simulink library "lib_imuCal"  (Simulink 9.0)
settings: Solver=VariableStepAuto  StartTime=0.0  StopTime=10.0  RelTol=1e-3
undefined symbols (not defined in the file): g, toa_imuBasicOrient
libraries: lib_CATutils_Utilities_ApplyName_v2 x14, lib_imuCal x2, simulink_extras x2, lib_CATutils_Override x2
(part 2 of 2)

== matlab function imuCal Subsystem/imuCal ==
  data: resetLowerFlag input double; pitchOffset output double; resetRaiseFlag input double; calDirectionFlag input double; getPitchOffsetFlag input double; liftHeight input double; tiltHePress input double; tiltRePress input double; liftPress input double; imuX input double; imuY input double; imuZ input double; liftAngle input double; tiltExt input double; steerAngle input double; toa_appNumber input double; toa_tiltBoreDia input double; toa_tiltRodDia input double; toa_liftBoreDia input double; toa_tiltNumCyl input double; toa_toolBcLength input double; lumpedWeight output double
function [pitchOffset, lumpedWeight] = imuCal(...
    resetLowerFlag, resetRaiseFlag, calDirectionFlag, getPitchOffsetFlag, ...
    liftHeight, tiltHePress, tiltRePress, liftPress, ...
    imuX, imuY, imuZ, ...
    liftAngle, tiltExt, steerAngle, ...
    toa_appNumber, toa_tiltBoreDia, toa_tiltRodDia, toa_liftBoreDia, toa_tiltNumCyl, toa_toolBcLength)
% IMUCAL Calibrate IMU
%
% Collects data during CPM calibration and calculates an IMU pitch offset
% calibration value.
%
% Data is collected between the *_TRIGGER_HEIGHT lift heights during the
% slow loaded raise and slow loaded lower portion of the CPM cal.  Then, a
% brute force search for the correct IMU pitch cal value begins.  For
% candidate pitch values (which are an input into the TOA weighing math,
% the following occurs.
%
% Tip-Off Assist weighing math is applied to obtain a corresponding weight
% signal for both raise a lower.  The signals include friction.  A
% phaseless notch filter is applied to the weight signals to remove machine
% resonance. The raise and lower weight signals are then sampled at the
% lift angles specified by *_LA_SLOPE_POINTS.  The weights at the sample
% points are averaged to produce a frictionless weight at each lift angle.
% Finally, the slope of the lift angle vs. frictionless weight curve is
% calculated.
%
% The correct IMU pitch cal value will be the one whose corresponding slope
% is closest to zero, because the correct cal value should produce the same
% weight across the lift range.

% To enable some code paths that may be useful for development.
DEBUG = false;

% Sample time
% Important for phaseless filtering
Ts = single(0.020);

% Constants
% Slope points a grid of lift angles (in degrees) that we sample the
% time-series data to for purposes of calculating slope efficiently.  This
% is done after phaseless filtering.
LA_SLOPE_POINTS_BOTTOM = -10;   % MUST be higher than BOTTOM_TRIGGER_HEIGHT
LA_SLOPE_POINTS_TOP = 15;       % MUST be lower than TOP_TRIGGER_HEIGHT
LA_SLOPE_POINTS_INC = 0.5;
LA_SLOPE_POINTS_NUM = (LA_SLOPE_POINTS_TOP - LA_SLOPE_POINTS_BOTTOM) / LA_SLOPE_POINTS_INC + 1;
LA_SLOPE_POINTS_IDX_NEW = zeros(1, LA_SLOPE_POINTS_NUM);
RAISE_LA_SLOPE_POINTS = LA_SLOPE_POINTS_BOTTOM : LA_SLOPE_POINTS_INC : LA_SLOPE_POINTS_TOP;
LOWER_LA_SLOPE_POINTS = LA_SLOPE_POINTS_TOP : -LA_SLOPE_POINTS_INC : LA_SLOPE_POINTS_BOTTOM;
BOTTOM_TRIGGER_HEIGHT = 35; % MUST be lower than LA_SLOPE_POINTS_BOTTOM
TOP_TRIGGER_HEIGHT = 80;    % MUST be heigher than LA_SLOPE_POINTS_TOP
RAISE_START_HEIGHT = BOTTOM_TRIGGER_HEIGHT;
RAISE_END_HEIGHT = TOP_TRIGGER_HEIGHT;
LOWER_START_HEIGHT = TOP_TRIGGER_HEIGHT;
LOWER_END_HEIGHT = BOTTOM_TRIGGER_HEIGHT;
MAX_CAPTURE_TIME = 55;  % seconds per raise or lower
BUFFER_LEN = MAX_CAPTURE_TIME / Ts;
NEW_BUFFER = single(zeros(1, BUFFER_LEN));
SEARCH_MIN = single(-8);
SEARCH_MAX = single(8);
SEARCH_INCREMENT = single(0.1);
SEARCH_SPACE_SIZE = (SEARCH_MAX - SEARCH_MIN) / SEARCH_INCREMENT + 1;
SEARCH_PITCH_OFFSETS = SEARCH_MIN : SEARCH_INCREMENT : SEARCH_MAX;

% Variables that will persist across function calls
persistent initialized

persistent lowerStarted
persistent lowerDone
persistent lowerFailed
persistent lowerBufferIdx
persistent lowerLaSlopePointsDone
persistent lowerLaSlopePointsIdxs
persistent lowerLaSlopePointsIdx
persistent lowerBufTiltHePress
persistent lowerBufTiltRePress
persistent lowerBufLiftPress
persistent lowerBufImuX
persistent lowerBufImuY
persistent lowerBufImuZ
persistent lowerBufLiftAngle
persistent lowerBufTiltExt
persistent lowerBufSteerAngle

persistent raiseStarted
persistent raiseDone
persistent raiseFailed
persistent raiseBufferIdx
persistent raiseLaSlopePointsDone
persistent raiseLaSlopePointsIdxs
persistent raiseLaSlopePointsIdx
persistent raiseBufTiltHePress
persistent raiseBufTiltRePress
persistent raiseBufLiftPress
persistent raiseBufImuX
persistent raiseBufImuY
persistent raiseBufImuZ
persistent raiseBufLiftAngle
persistent raiseBufTiltExt
persistent raiseBufSteerAngle

% Initialize persistent variables
if isempty(initialized)
    initialized = 1;
    % Raise
    raiseStarted = false;
    raiseDone = false;
    raiseFailed = false;
    raiseBufferIdx = 0;
    raiseLaSlopePointsDone = false;
    raiseLaSlopePointsIdxs = LA_SLOPE_POINTS_IDX_NEW;
    raiseLaSlopePointsIdx = 1;
    raiseBufTiltHePress = NEW_BUFFER;
    raiseBufTiltRePress = NEW_BUFFER;
    raiseBufLiftPress = NEW_BUFFER;
    raiseBufImuX = NEW_BUFFER;
    raiseBufImuY = NEW_BUFFER;
    raiseBufImuZ = NEW_BUFFER;
    raiseBufLiftAngle = NEW_BUFFER;
    raiseBufTiltExt = NEW_BUFFER;
    raiseBufSteerAngle = NEW_BUFFER;
    % Lower
    lowerStarted = false;
    lowerDone = false;
    lowerFailed = false;
    lowerBufferIdx = 0;
    lowerLaSlopePointsDone = false;
    lowerLaSlopePointsIdxs = LA_SLOPE_POINTS_IDX_NEW;
    lowerLaSlopePointsIdx = 1;
    lowerBufTiltHePress = NEW_BUFFER;
    lowerBufTiltRePress = NEW_BUFFER;
    lowerBufLiftPress = NEW_BUFFER;
    lowerBufImuX = NEW_BUFFER;
    lowerBufImuY = NEW_BUFFER;
    lowerBufImuZ = NEW_BUFFER;
    lowerBufLiftAngle = NEW_BUFFER;
    lowerBufTiltExt = NEW_BUFFER;
    lowerBufSteerAngle = NEW_BUFFER;

end

% Reset procedure
if resetLowerFlag || resetRaiseFlag
    fprintf('# RESET - imuCal() called with arguments:\n')
    fprintf('## resetLowerFlag = %u\n', uint8(resetLowerFlag))
    fprintf('## resetRaiseFlag = %u\n', uint8(resetRaiseFlag))
    fprintf('## calDirectionFlag = %u\n', uint8(calDirectionFlag))
    fprintf('## getPitchOffsetFlag = %u\n', uint8(getPitchOffsetFlag))
    if resetLowerFlag
        lowerStarted = false;
        lowerDone = false;
        lowerFailed = false;
        lowerBufferIdx = 0;
        lowerLaSlopePointsDone = false;
        lowerLaSlopePointsIdxs = LA_SLOPE_POINTS_IDX_NEW;
        lowerLaSlopePointsIdx = 1;
        lowerBufTiltHePress = NEW_BUFFER;
        lowerBufTiltRePress = NEW_BUFFER;
        lowerBufLiftPress = NEW_BUFFER;
        lowerBufImuX = NEW_BUFFER;
        lowerBufImuY = NEW_BUFFER;
        lowerBufImuZ = NEW_BUFFER;
        lowerBufLiftAngle = NEW_BUFFER;
        lowerBufTiltExt = NEW_BUFFER;
        lowerBufSteerAngle = NEW_BUFFER;
    end
    if resetRaiseFlag
        raiseStarted = false;
        raiseDone = false;
        raiseFailed = false;
        raiseBufferIdx = 0;
        raiseLaSlopePointsDone = false;
        raiseLaSlopePointsIdxs = LA_SLOPE_POINTS_IDX_NEW;
        raiseLaSlopePointsIdx = 1;
        raiseBufTiltHePress = NEW_BUFFER;
        raiseBufTiltRePress = NEW_BUFFER;
        raiseBufLiftPress = NEW_BUFFER;
        raiseBufImuX = NEW_BUFFER;
        raiseBufImuY = NEW_BUFFER;
        raiseBufImuZ = NEW_BUFFER;
        raiseBufLiftAngle = NEW_BUFFER;
        raiseBufTiltExt = NEW_BUFFER;
        raiseBufSteerAngle = NEW_BUFFER;
    end
    pitchOffset = single(NaN);
    lumpedWeight = single(NaN);
    return
end

% Pitch Calibration Procedure
% Brute-force search for flattest height vs. weight curve
if getPitchOffsetFlag
    fprintf('# GET OFFSET - imuCal() called with arguments:\n')
    fprintf('## resetLowerFlag = %u\n', uint8(resetLowerFlag))
    fprintf('## resetRaiseFlag = %u\n', uint8(resetRaiseFlag))
    fprintf('## calDirectionFlag = %u\n', uint8(calDirectionFlag))
    fprintf('## getPitchOffsetFlag = %u\n', uint8(getPitchOffsetFlag))
    fprintf('### RAISE\n')
    fprintf('#### raiseBufferIdx = %u\n', uint8(raiseBufferIdx))
    fprintf('#### raiseFailed = %u\n', uint8(raiseFailed))
    fprintf('#### raiseStarted = %u\n', uint8(raiseStarted))
    fprintf('#### raiseDone = %u\n', uint8(raiseDone))
    fprintf('#### lift angle min = %.1f, max = %.1f\n', min(raiseBufLiftAngle), max(raiseBufLiftAngle))
    fprintf('### LOWER\n')
    fprintf('#### lowerBufferIdx = %u\n', uint8(lowerBufferIdx))
    fprintf('#### lowerFailed = %u\n', uint8(lowerFailed))
    fprintf('#### lowerStarted = %u\n', uint8(lowerStarted))
    fprintf('#### lowerDone = %u\n', uint8(lowerDone))
    fprintf('#### lift angle min = %.1f, max = %.1f\n', min(lowerBufLiftAngle), max(lowerBufLiftAngle))
    if raiseFailed || lowerFailed
        pitchOffset = single(NaN);
        lumpedWeight = single(NaN);
        fprintf('Raise or lower failed.  getPitchOffset not possible.')
        return
    end
    % Allocate buffers of brute-force search calculated weights
    searchRaiseSlopes = zeros(SEARCH_SPACE_SIZE, 1);
    searchLowerSlopes = zeros(SEARCH_SPACE_SIZE, 1);
    searchNoFricSlopes = zeros(SEARCH_SPACE_SIZE, 1);
    searchLeastSlope = single(9999);
    searchLeastSlopeIdx = single(999999);
    searchLeastSlopePitchOffset = single(NaN);
    searchLeastSlopeLumpedWeight = single(NaN);
    for searchIdx = 1:SEARCH_SPACE_SIZE
        searchPitchOffset = SEARCH_PITCH_OFFSETS(searchIdx);
        if DEBUG
            if raiseDone
                searchRaiseSlopes(searchIdx, 1) = getSlope(...
                    raiseLaSlopePointsIdxs,...
                    raiseBufferIdx,...
                    Ts,...
                    raiseBufLiftAngle,...
                    raiseBufTiltExt,...
                    raiseBufTiltHePress,...
                    raiseBufTiltRePress,...
                    raiseBufLiftPress,...
                    raiseBufImuX,...
                    raiseBufImuY,...
                    raiseBufImuZ,...
                    raiseBufSteerAngle,...
                    searchPitchOffset,...
                    searchIdx,...
                    toa_appNumber, toa_tiltBoreDia, toa_tiltRodDia, toa_liftBoreDia, toa_tiltNumCyl, toa_toolBcLength...
                );
            end
            if lowerDone
                searchLowerSlopes(searchIdx, 1) = getSlope(...
                    lowerLaSlopePointsIdxs,...
                    lowerBufferIdx,...
                    Ts,...
                    lowerBufLiftAngle,...
                    lowerBufTiltExt,...
                    lowerBufTiltHePress,...
                    lowerBufTiltRePress,...
                    lowerBufLiftPress,...
                    lowerBufImuX,...
                    lowerBufImuY,...
                    lowerBufImuZ,...
                    lowerBufSteerAngle,...
                    searchPitchOffset,...
                    searchIdx,...
                    toa_appNumber, toa_tiltBoreDia, toa_tiltRodDia, toa_liftBoreDia, toa_tiltNumCyl, toa_toolBcLength...
                );
            end
        end
        if lowerDone && raiseDone
            searchRaiseWeight = calcMass(...
                raiseBufferIdx,...
                Ts,...
                raiseBufLiftAngle,...
                raiseBufTiltExt,...
                raiseBufTiltHePress,...
                raiseBufTiltRePress,...
                raiseBufLiftPress,...
                raiseBufImuX,...
                raiseBufImuY,...
                raiseBufImuZ,...
                raiseBufSteerAngle,...
                searchPitchOffset,...
                toa_appNumber, toa_tiltBoreDia, toa_tiltRodDia, toa_liftBoreDia, toa_tiltNumCyl, toa_toolBcLength...
            );
            searchLowerWeight = calcMass(...
                lowerBufferIdx,...
                Ts,...
                lowerBufLiftAngle,...
                lowerBufTiltExt,...
                lowerBufTiltHePress,...
                lowerBufTiltRePress,...
                lowerBufLiftPress,...
                lowerBufImuX,...
                lowerBufImuY,...
                lowerBufImuZ,...
                lowerBufSteerAngle,...
                searchPitchOffset,...
                toa_appNumber, toa_tiltBoreDia, toa_tiltRodDia, toa_liftBoreDia, toa_tiltNumCyl, toa_toolBcLength...
            );
            searchNoFricWeight = (searchRaiseWeight(raiseLaSlopePointsIdxs) + searchLowerWeight(fliplr(lowerLaSlopePointsIdxs))) / 2;
            dummy = polyfit(RAISE_LA_SLOPE_POINTS, searchNoFricWeight, 1);
            searchNoFricSlope = dummy(1);
            searchNoFricSlopes(searchIdx) = searchNoFricSlope;
            if abs(searchNoFricSlope) < abs(searchLeastSlope)
                searchLeastSlope = searchNoFricSlope;
                searchLeastSlopeIdx = searchIdx;
                searchLeastSlopePitchOffset = searchPitchOffset;
                searchLeastSlopeLumpedWeight = mean(searchNoFricWeight);
            end
        end
    end
    
    % Calculate results and print them
    if DEBUG
        if raiseDone
            [dummy, raiseFlattestSlopeSearchIdx] = min(abs(searchRaiseSlopes));
            raiseFlattestSlope = searchRaiseSlopes(raiseFlattestSlopeSearchIdx);
            raisePitchOffset = SEARCH_PITCH_OFFSETS(raiseFlattestSlopeSearchIdx);
            disp('# Raise Pitch Result #')
            fprintf('## Slope = %.4f\n## Index = %f\n## Pitch = %.4f\n', raiseFlattestSlope, raiseFlattestSlopeSearchIdx, raisePitchOffset)
            disp(raisePitchOffset)
        else
            raisePitchOffset = single(NaN);
        end

        if lowerDone
            [dummy, lowerFlattestSlopeSearchIdx] = min(abs(searchLowerSlopes));
            lowerFlattestSlope = searchLowerSlopes(lowerFlattestSlopeSearchIdx);
            lowerPitchOffset = SEARCH_PITCH_OFFSETS(lowerFlattestSlopeSearchIdx);
            disp('# Lower Pitch Result #')
            fprintf('## Slope = %.4f\n## Index = %f\n## Pitch = %.4f\n', lowerFlattestSlope, lowerFlattestSlopeSearchIdx, lowerPitchOffset)
            disp(lowerPitchOffset)
        else
            lowerPitchOffset = single(NaN);
        end
    end
    
    if raiseDone && lowerDone
        disp('# Frictionless Pitch Result #')
        fprintf('## Slope = %.4f\n## Index = %f\n## Pitch = %.4f\n## Weight = %.4f\n', searchLeastSlope, searchLeastSlopeIdx, searchLeastSlopePitchOffset, searchLeastSlopeLumpedWeight)
        disp(searchLeastSlopePitchOffset)
    end
    
    % Set return value and return
    if raiseDone && lowerDone
        pitchOffset = searchLeastSlopePitchOffset;
        lumpedWeight = searchLeastSlopeLumpedWeight;
    else
        pitchOffset = single(NaN);
        lumpedWeight = single(NaN);
    end
    fprintf('# Returned Pitch Offset = %.4f\n', pitchOffset);
    return
end

% Data Collection - Raise
if calDirectionFlag == 0 % Raise
    if raiseBufferIdx == BUFFER_LEN
        fprintf('IMU Cal: Raise data capture failed due to buffer too small!\n');
        raiseFailed = true;
    end
    if liftHeight > RAISE_START_HEIGHT
        raiseStarted = true;
    end
    if liftHeight > RAISE_END_HEIGHT
        raiseDone = true;
    end
    if raiseStarted && ~raiseDone && ~raiseFailed
        raiseBufferIdx = raiseBufferIdx + 1;
        raiseBufTiltHePress(raiseBufferIdx) = tiltHePress;
        raiseBufTiltRePress(raiseBufferIdx) = tiltRePress;
        raiseBufLiftPress(raiseBufferIdx) = liftPress;
        raiseBufImuX(raiseBufferIdx) = imuX;
        raiseBufImuY(raiseBufferIdx) = imuY;
        raiseBufImuZ(raiseBufferIdx) = imuZ;
        raiseBufLiftAngle(raiseBufferIdx) = liftAngle;
        raiseBufTiltExt(raiseBufferIdx) = tiltExt;
        raiseBufSteerAngle(raiseBufferIdx) = steerAngle;
        
        if ~raiseLaSlopePointsDone && liftAngle > RAISE_LA_SLOPE_POINTS(raiseLaSlopePointsIdx)
            raiseLaSlopePointsIdxs(raiseLaSlopePointsIdx) = raiseBufferIdx;
            if raiseLaSlopePointsIdx < LA_SLOPE_POINTS_NUM
                raiseLaSlopePointsIdx = raiseLaSlopePointsIdx + 1;
                if liftAngle > RAISE_LA_SLOPE_POINTS(raiseLaSlopePointsIdx)
                    % Already passed next slope point unexpectedly
                    raiseFailed = true;
                    fprintf('IMU Cal: Raise data capture failed due to func not called frequently enough!\n');
                end
            else
                raiseLaSlopePointsDone = true;
            end
        end
    end
    pitchOffset = single(NaN);
    lumpedWeight = single(NaN);
    return
end

% Data Collection - Lower
if calDirectionFlag == 1 % Lower
    if lowerBufferIdx == BUFFER_LEN
        fprintf('IMU Cal: Lower data capture failed due to buffer too small!\n');
        lowerFailed = true;
    end
    if liftHeight < LOWER_START_HEIGHT
        lowerStarted = true;
    end
    if liftHeight < LOWER_END_HEIGHT
        lowerDone = true;
    end
    if lowerStarted && ~lowerDone && ~lowerFailed
        lowerBufferIdx = lowerBufferIdx + 1;
        lowerBufTiltHePress(lowerBufferIdx) = tiltHePress;
        lowerBufTiltRePress(lowerBufferIdx) = tiltRePress;
        lowerBufLiftPress(lowerBufferIdx) = liftPress;
        lowerBufImuX(lowerBufferIdx) = imuX;
        lowerBufImuY(lowerBufferIdx) = imuY;
        lowerBufImuZ(lowerBufferIdx) = imuZ;
        lowerBufLiftAngle(lowerBufferIdx) = liftAngle;
        lowerBufTiltExt(lowerBufferIdx) = tiltExt;
        lowerBufSteerAngle(lowerBufferIdx) = steerAngle;
        
        if ~lowerLaSlopePointsDone && liftAngle < LOWER_LA_SLOPE_POINTS(lowerLaSlopePointsIdx)
            lowerLaSlopePointsIdxs(lowerLaSlopePointsIdx) = lowerBufferIdx;
            if lowerLaSlopePointsIdx < LA_SLOPE_POINTS_NUM
                lowerLaSlopePointsIdx = lowerLaSlopePointsIdx + 1;
                if liftAngle < LOWER_LA_SLOPE_POINTS(lowerLaSlopePointsIdx)
                    % Already passed next slope point unexpectedly
                    lowerFailed = true;
                    fprintf('IMU Cal: Lower data capture failed due to func not called frequently enough!\n');
                end
            else
                lowerLaSlopePointsDone = true;
            end
        end
    end
    pitchOffset = single(NaN);
    lumpedWeight = single(NaN);
    return
end

% We should never get down here
pitchOffset = single(NaN);
lumpedWeight = single(NaN);
return

    function slope = getSlope(laSlopePointIdxs, endDataIdx, Ts, bufLiftAngle, bufTiltExt, bufTiltHePress, bufTiltRePress, bufLiftPress, bufImuX, bufImuY, bufImuZ, bufSteerAngle, pitchOffset, searchIdx, ...
                              toa_appNumber, toa_tiltBoreDia, toa_tiltRodDia, toa_liftBoreDia, toa_tiltNumCyl, toa_toolBcLength)
        % Calculates raw TOA weight and filters it with a phaseless notch
        % filter. Then, calculates the slope of lift angle vs. weight, as
        % sampled at the LA slope points.
        z = searchIdx;
        bufferLen = length(bufLiftAngle);
        weights = single(zeros(1, bufferLen));
        weightsFilt = single(zeros(1, bufferLen));
        phaselessTemp = single(zeros(1, bufferLen));
        slopePointWeightsFilt = single(zeros(1, 21));
        slopePointsLiftAngles = single(zeros(1, 21));
        for idx = 1:endDataIdx
            weights(idx) = toa_imuCalPayload(...
                    bufLiftAngle(idx),...
                    bufTiltExt(idx),...
                    bufTiltHePress(idx),...
                    bufTiltRePress(idx),...
                    bufLiftPress(idx),...
                    bufImuX(idx),...
                    bufImuY(idx),...
                    bufImuZ(idx),...
                    bufSteerAngle(idx),...
                    pitchOffset,...
                    toa_appNumber, toa_tiltBoreDia, toa_tiltRodDia, toa_liftBoreDia, toa_tiltNumCyl, toa_toolBcLength...
            );
            if idx == 1
                dummy = notchFilter(weights(idx), true, Ts);  %reset filter
            end
            phaselessTemp(idx) = notchFilter(weights(idx), false, Ts);
        end
        dummy = notchFilter(phaselessTemp(endDataIdx), true, Ts);   %reset filter to prepare for reverse pass
        for idx = 1:endDataIdx
            reverseIdx = endDataIdx - idx + 1;
            weightsFilt(reverseIdx) = notchFilter(phaselessTemp(reverseIdx), false, Ts);
        end
        for spIdx = 1:21
            slopePointsLiftAngles(spIdx) = bufLiftAngle(laSlopePointIdxs(spIdx));
            slopePointWeightsFilt(spIdx) = weightsFilt(laSlopePointIdxs(spIdx));
        end
        dummy = polyfit(slopePointsLiftAngles, slopePointWeightsFilt, 1);
        slope = dummy(1);
        return
        
    function weightsFilt = calcMass(endDataIdx, Ts, bufLiftAngle, bufTiltExt, bufTiltHePress, bufTiltRePress, bufLiftPress, bufImuX, bufImuY, bufImuZ, bufSteerAngle, pitchOffset, ...
                                    toa_appNumber, toa_tiltBoreDia, toa_tiltRodDia, toa_liftBoreDia, toa_tiltNumCyl, toa_toolBcLength)
        % Calculates raw TOA weight and filters it with a phaseless notch
        % filter.
        bufferLen = length(bufLiftAngle);
        weights = single(zeros(1, bufferLen));
        weightsFilt = single(zeros(1, bufferLen));
        phaselessTemp = single(zeros(1, bufferLen));
        for idx = 1:endDataIdx
            weights(idx) = toa_imuCalPayload(...
                    bufLiftAngle(idx),...
                    bufTiltExt(idx),...
                    bufTiltHePress(idx),...
                    bufTiltRePress(idx),...
                    bufLiftPress(idx),...
                    bufImuX(idx),...
                    bufImuY(idx),...
                    bufImuZ(idx),...
                    bufSteerAngle(idx),...
                    pitchOffset,...
                    toa_appNumber, toa_tiltBoreDia, toa_tiltRodDia, toa_liftBoreDia, toa_tiltNumCyl, toa_toolBcLength...
            );
            if idx == 1
                dummy = notchFilter(weights(idx), true, Ts);  %reset filter to prepare for forward pass
            end
            phaselessTemp(idx) = notchFilter(weights(idx), false, Ts);
        end
        dummy = notchFilter(phaselessTemp(endDataIdx), true, Ts);   %reset filter to prepare for reverse pass
        for idx = 1:endDataIdx
            reverseIdx = endDataIdx - idx + 1;
            weightsFilt(reverseIdx) = notchFilter(phaselessTemp(reverseIdx), false, Ts);
        end
        
        return

== matlab function imuCal Subsystem/TOA Weight Simulink Function/EEF IMU to NEEF gravity vector/euler angles from rot matrix ==
  data: rotations output double; rotMatrix input double
function rotations  = decomp(rotMatrix)
%   Input:  3x3 rotation matrix
%   Output: 1x3 vector of euler angles in degrees
rotations = zeros(1,3);
rotations(1) = atan2(rotMatrix(3,2),rotMatrix(3,3));
rotations(2) = atan2(-rotMatrix(3,1), (sqrt((rotMatrix(3,2)^2)+(rotMatrix(3,3)^2))));
rotations(3) = atan2(rotMatrix(2,1),rotMatrix(1,1));
% convert back to degrees
for i=1:size(rotations,2)
    rotations(i) = 180*rotations(i)/pi;
end
end

== matlab function imuCal Subsystem/TOA Weight Simulink Function/EEF IMU to NEEF gravity vector/rotation matrix calc from two vectors ==
  data: level_vec_meas input double; rotMatrix output double; level_vec_act input double; rotAxis output double; angle output double
function [rotMatrix, rotAxis, angle] = fcn(level_vec_meas, level_vec_act)
% Should match output of:
%     vrrotvec2mat(vrrotvec(level_vec_meas, level_vec_act))

if all(level_vec_meas == level_vec_act)
    % No transform necessary, return identity matrix
    rotAxis = single([9999; 9999; 9999]);
    angle = single(9999);
    rotMatrix = single(eye(3));
    return
end
    
a = level_vec_meas;
b = level_vec_act;

cp = cross(a, b);
cpNorm = norm(cp);

rotAxis = cp/cpNorm;
angle_rad = atan(cpNorm/dot(a, b));
angle = angle_rad * 180.0 / pi;

% Form rotation matrix
crossProductMatrix = [
    0,          -rotAxis(3),  rotAxis(2);
     rotAxis(3), 0,          -rotAxis(1);
    -rotAxis(2), rotAxis(1),  0
];
tensorProduct = rotAxis * transpose(rotAxis);
rotMatrix = cos(angle_rad) * eye(3) + sin(angle_rad) * crossProductMatrix + ...
    (1 - cos(angle_rad)) * tensorProduct;
